simulink model "speed_controller_discrete"  (R2025b)
settings: Solver=FixedStepDiscrete  FixedStep=speedControl.sampleTime_s
undefined symbols (not defined in the file): DiscIntNeverNeededParam, speedControl
settings Model: Creator=Semih  LastModifiedBy=Semih
settings SFSimCC: SimGPUStackLimitPerThread=51200  SimGPUMallocThreshold=200
settings RTWCC: GPUStackLimitPerThread=51200  GPUMallocThreshold=200

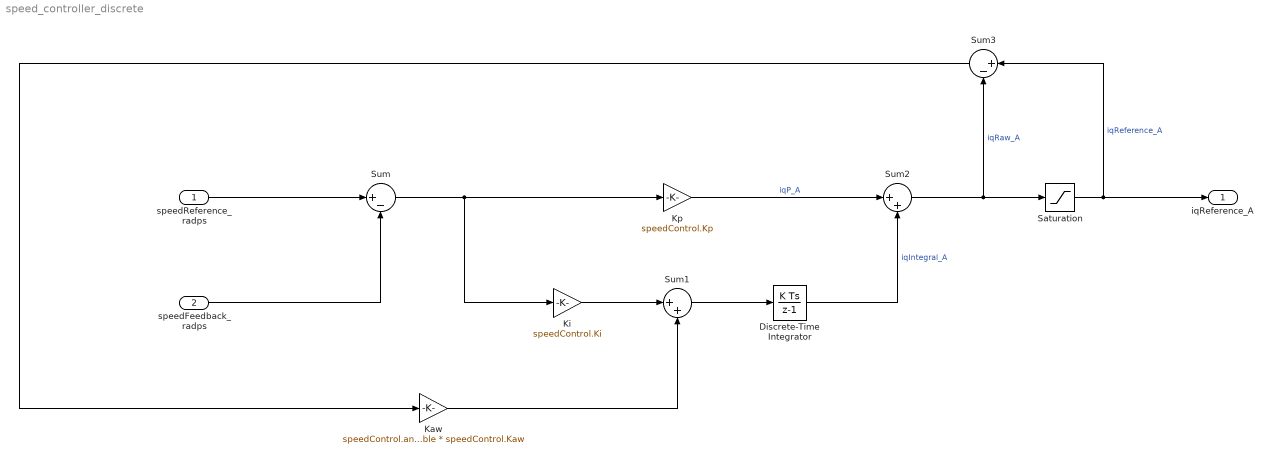
== system speed_controller_discrete ==
  speedReference_radps : Inport
  speedFeedback_radps : Inport  Port=2
  Discrete-Time Integrator : DiscreteIntegrator  SampleTime=speedControl.sampleTime_s  ICPrevOutput=DiscIntNeverNeededParam  ICPrevScaledInput=DiscIntNeverNeededParam
  Kaw : Gain  Gain=speedControl.antiWindupEnable * speedControl.Kaw
  Ki : Gain  Gain=speedControl.Ki
  Kp : Gain  Gain=speedControl.Kp
  Saturation : Saturate  UpperLimit=speedControl.iqLimit_A  LowerLimit=-speedControl.iqLimit_A
  Sum : Sum  Inputs=|+-
  Sum1 : Sum  Inputs=|++
  Sum2 : Sum  Inputs=|++
  Sum3 : Sum  Inputs=|+-
  iqReference_A : Outport
  wires:
  speedReference_radps/1 -> Sum/1
  speedFeedback_radps/1 -> Sum/2
  Sum/1 -> Ki/1, Kp/1
  Ki/1 -> Sum1/1
  Sum3/1 -> Kaw/1
  Kaw/1 -> Sum1/2
  Sum1/1 -> Discrete-Time Integrator/1
  Discrete-Time Integrator/1 -> Sum2/2  "iqIntegral_A"
  Kp/1 -> Sum2/1  "iqP_A"
  Sum2/1 -> Saturation/1, Sum3/2  "iqRaw_A"
  Saturation/1 -> Sum3/1, iqReference_A/1  "iqReference_A"
